simulink model "sptr"  (R2026a)
settings: Solver=daessc  StopTime=simlength  FixedStep=Ts  MaxStep=Ts  RelTol=Ts  AbsTol=Ts  EnableMultiTasking=on
values from neighbouring files (symbols this model uses):
  I_FS = Iout_dc_nom * margin_factor    (= 103.5)    [init_model.m]
  kgrid = 1    [init_model.m]
  LFu_dc = 1.2e-3    (= 0.0012)    [init_model.m]
  pll_i1 = 80    [init_model.m]
  pll_p = 1    [init_model.m]
  RLFu_dc = 2e-4    (= 0.0002)    [init_model.m]
  Rload = 1.2/4    (= 0.3)    [init_model.m]
  Tcontrol_rect = tPWM_RECT    (= 0.0002)    [init_model.m]
  Ts = Tc/1    (= 1e-05)    [init_model.m]
  V_FS = Vout_dc_nom * margin_factor    (= 391)    [init_model.m]
  Vnom_ac_adc = 400/sqrt(3)*sqrt(2)    [init_model.m]
  Vphase1 = Vline1/sqrt(3)    [init_model.m]
  w_grid = f_grid*2*pi    (= 314.159265359)    [init_model.m]
undefined symbols (not defined in the file or in its folder): magnitude
libraries: fl_lib x137, nesl_utility x33, ee_lib x15, first_harmonic_tracker x3
(part 1 of 3)
settings Model: SimulationMode=accelerator  Creator=LTNBDA  LastModifiedBy=dbagn
settings SolverCC: ZeroCrossControl=EnableAll  ZeroCrossAlgorithm=Adaptive  SolverResetMethod=Robust
settings DataIOCC: MaxDataPoints=1  SignalLoggingSaveFormat=ModelDataLogs
settings OptimizationCC: InitFltsAndDblsToZero=on  EfficientMapNaN2IntZero=off
settings DebuggingCC: SaveWithParameterizedLinksMsg=none  SignalResolutionControl=TryResolveAllWithWarning  MultiTaskDSMMsg=warning  MultiTaskCondExecSysMsg=none
settings HardwareCC: ProdBitPerLong=64.0  ProdHWDeviceType=Generic->64-bit Embedded Processor (LP64)  TargetBitPerPointer=64.0  TargetBitPerSizeT=64.0  TargetBitPerPtrDiffT=64.0  TargetLongLongMode=on  TargetIntDivRoundTo=Zero  TargetEndianess=LittleEndian  TargetWordSize=64.0  TargetHWDeviceType=MATLAB Host  ProdEqTarget=off
settings SFSimCC: SimCustomHeaderCode=|
  | #include "math_f.h"
  | #include "mavgflt.h"
  | #include "mavgflt_simulink.h"
  | #include "bemf_obsv.h"
  | #include "bemf_obsv_simulink.h"
  | #include "bemf_obsv_load_est.h"
  | #include "bemf_obsv_load_est_simulink.h"
  | #include "dqvector_pi.h"
  | #include "dqvector_pi_simulink.h"
  | #include "sv_pwm_simulink.h"
  | #include "sv_pwm.h"
  | #include "six_pulse_rect.h"
  | #include "twelve_pulse_rect.h"
  | #include "first_harmonic_tracker.h"
  | #include "first_harmonic_tracker_simulink.h"
  | #include "dqpll_thyr.h"
  | #include "dqpll_thyr_simulink.h"
  | #include "dqpll_grid.h"
  | #include "dqpll_grid_simulink.h"
settings SFSimCC: SimUserSources=|
  | "mavgflt_simulink.c"
  | "mavgflt.c"
  | "bemf_obsv_simulink.c"
  | "bemf_obsv.c"
  | "bemf_obsv_load_est_simulink.c"
  | "bemf_obsv_load_est.c"
  | "dqvector_pi.c"
  | "dqvector_pi_simulink.c"
  | "sv_pwm_simulink.c"
  | "sv_pwm.c"
  | "six_pulse_rect.c"
  | "twelve_pulse_rect.c"
  | "first_harmonic_tracker_simulink.c"
  | "first_harmonic_tracker.c"
  | "dqpll_thyr_simulink.c"
  | "dqpll_thyr.c"
  | "dqpll_grid_simulink.c"
  | "dqpll_grid.c"
settings SFSimCC: SimUserIncludeDirs=|
  | include
  | src
settings CodeAppCC: MaxIdLength=128.0
settings GRTTargetCC: CombineOutputUpdateFcns=off  GRTInterface=on
settings SimscapeCC: SimscapeNormalizeSystem=off  SimscapeNominalValues="[{\"value\":\"1\",\"unit\":\"A\"},{\"value\":\"1\",\"unit\":\"bar\"},{\"value\":\"1\",\"unit\":\"cm^2\"},{\"value\":\"1\",\"unit\":\"cm^3/s\"},{\"value\":\"1\",\"unit\":\"kJ/kg\"},{\"value\":\"1\",\"unit\":\"kW\"},{\"value\":\"1\",\"unit\":\"l\"},{\"value\":\"1\",\"unit\":\"N\"},{\"value\":\"1\",\"unit\":\"N*m\"},{\"value\":\"1\",\"unit\":\"V\"}]"  SimscapeLogType=none  SimscapeLogDataHistory=5000.0

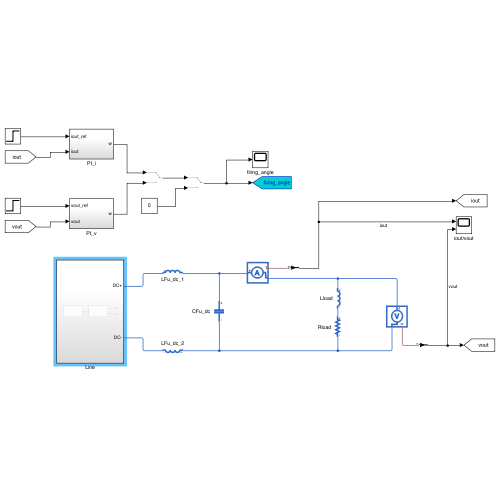
[thumbnail: Simulink's stored preview of the top-level diagram]
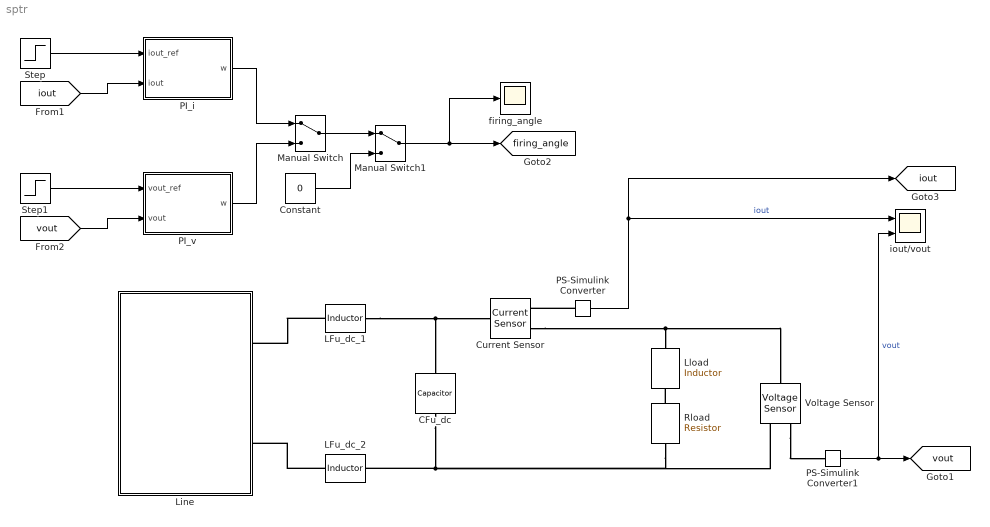
== system sptr ==
  CFu_dc : fl_lib/Electrical/Electrical Elements/Capacitor  c=CFu_dc F  r=RCFu_dc Ohm  g=0 1/Ohm  i_specify=off  i_priority=None  i=0 A  i_nominal_specify=off  i_nominal_value=1  i_nominal_unit=A  v_specify=off  v_priority=None  v=0 V  v_nominal_specify=off  v_nominal_value=1  v_nominal_unit=V  vc_specify=off  vc_priority=High  vc=0 V  vc_nominal_specify=off  vc_nominal_value=1  vc_nominal_unit=V
  Constant : Constant  Value=0
  Current Sensor : fl_lib/Electrical/Electrical Sensors/Current Sensor
  LFu_dc_1 : fl_lib/Electrical/Electrical Elements/Inductor  l=LFu_dc/2 H  r=RLFu_dc/2 Ohm  g=1e-9 1/Ohm  i_specify=off  i_priority=None  i=0 A  i_nominal_specify=off  i_nominal_value=1  i_nominal_unit=A  v_specify=off  v_priority=None  v=0 V  v_nominal_specify=off  v_nominal_value=1  v_nominal_unit=V  i_L_specify=off  i_L_priority=High  i_L=0 A  i_L_nominal_specify=off  i_L_nominal_value=1  i_L_nominal_unit=A
  LFu_dc_2 : fl_lib/Electrical/Electrical Elements/Inductor  l=LFu_dc/2 H  r=RLFu_dc/2 Ohm  g=1e-9 1/Ohm  i_specify=off  i_priority=None  i=0 A  i_nominal_specify=off  i_nominal_value=1  i_nominal_unit=A  v_specify=off  v_priority=None  v=0 V  v_nominal_specify=off  v_nominal_value=1  v_nominal_unit=V  i_L_specify=off  i_L_priority=High  i_L=0 A  i_L_nominal_specify=off  i_L_nominal_value=1  i_L_nominal_unit=A
  Line : Subsystem
  Lload : fl_lib/Electrical/Electrical Elements/Inductor  l=Lload H  r=0 Ohm  g=1e-9 1/Ohm  i_specify=off  i_priority=None  i=0 A  i_nominal_specify=off  i_nominal_value=1  i_nominal_unit=A  v_specify=off  v_priority=None  v=0 V  v_nominal_specify=off  v_nominal_value=1  v_nominal_unit=V  i_L_specify=off  i_L_priority=High  i_L=0 A  i_L_nominal_specify=off  i_L_nominal_value=1  i_L_nominal_unit=A
  Manual Switch : ManualSwitch
  Manual Switch1 : ManualSwitch
  PI_i : Subsystem
  PI_v : Subsystem
  PS-Simulink Converter : nesl_utility/PS-Simulink Converter  PhysicalDomain=network_engine_domain  SubClassName=ps_output  LeftPortType=input  RightPortType=output  PseudoPeriodic=off  Frequencies=[]  VectorFormat=1-D array  Unit=A  AffineConversion=off
  PS-Simulink Converter1 : nesl_utility/PS-Simulink Converter  PhysicalDomain=network_engine_domain  SubClassName=ps_output  LeftPortType=input  RightPortType=output  PseudoPeriodic=off  Frequencies=[]  VectorFormat=1-D array  Unit=V  AffineConversion=on
  Rload : fl_lib/Electrical/Electrical Elements/Resistor  R=Rload*2 Ohm  i_specify=off  i_priority=None  i=0 A  i_nominal_specify=off  i_nominal_value=1  i_nominal_unit=A  v_specify=off  v_priority=None  v=0 V  v_nominal_specify=off  v_nominal_value=1  v_nominal_unit=V
  Step : Step  Time=0.5  FinalValue=500/I_FS  SampleTime=0
  Step1 : Step  Time=0.5  FinalValue=200/V_FS  SampleTime=0
  Voltage Sensor : fl_lib/Electrical/Electrical Sensors/Voltage Sensor
  firing_angle : Scope
      settings: ActiveDisplayYMinimum=-0.39269908169872403  ActiveDisplayYMaximum=3.5342917352885173  DataLoggingVariableName=ScopeData5
  iout/vout : Scope  NumInputPorts=2
      settings: SampleTime=Tcontrol_rect  ActiveDisplayYMinimum=-109.3182  ActiveDisplayYMaximum=967.41622  DataLoggingVariableName=ScopeData10
  tag scope: firing_angle=global, iout=global, vout=global
  wires:
  PS-Simulink Converter/1 -> iout/vout/1, [iout]  "iout"
  Step/1 -> PI_i/1(iout_ref)
  PS-Simulink Converter1/1 -> iout/vout/2, [vout]  "vout"
  [iout] -> PI_i/2(iout)
  [vout] -> PI_v/2(vout)
  Step1/1 -> PI_v/1(vout_ref)
  PI_i/1(w) -> Manual Switch/1
  PI_v/1(w) -> Manual Switch/2
  Manual Switch/1 -> Manual Switch1/1
  Manual Switch1/1 -> firing_angle/1, [firing_angle]
  Constant/1 -> Manual Switch1/2
  connections:
  LFu_dc_1/RConn1 -- CFu_dc/LConn1 -- Current Sensor/LConn1
  CFu_dc/RConn1 -- Rload/RConn1 -- Voltage Sensor/RConn2 -- LFu_dc_2/LConn1
  LFu_dc_2/RConn1 -- Line/RConn2
  LFu_dc_1/LConn1 -- Line/RConn1
  Rload/LConn1 -- Lload/RConn1
  PS-Simulink Converter/LConn1 -- Current Sensor/RConn1
  Current Sensor/RConn2 -- Lload/LConn1 -- Voltage Sensor/LConn1
  Voltage Sensor/RConn1 -- PS-Simulink Converter1/LConn1

== system sptr/Line ==
  Grid : Subsystem
  six_pulse rectifier : Subsystem
  DC+ : PMIOPort  Side=Right
  DC- : PMIOPort  Port=2  Side=Right
  connections:
  six_pulse rectifier/RConn1 -- DC+/RConn1
  Grid/RConn1 -- six_pulse rectifier/LConn1
  six_pulse rectifier/RConn2 -- DC-/RConn1

== system sptr/PI_i ==
  iout_ref : Inport
  iout : Inport  Port=2
  1/Ti : Gain  Gain=0.15  SaturateOnIntegerOverflow=on  OutDataTypeStr=Inherit: Same as input  ParamDataTypeStr=Inherit: Same as input
  1/Ti2 : Gain  Gain=1/I_FS  SaturateOnIntegerOverflow=on  OutDataTypeStr=Inherit: Same as input  ParamDataTypeStr=Inherit: Same as input
  Saturation : Saturate  UpperLimit=pi  LowerLimit=0.1
  Saturation1 : Saturate  UpperLimit=1  LowerLimit=-1
  Sum1 : Sum  Inputs=+++  SaturateOnIntegerOverflow=on
  Sum2 : Sum  Inputs=+-  SaturateOnIntegerOverflow=on
  Sum3 : Sum  Inputs=-+  SaturateOnIntegerOverflow=on
  Trigonometric Function : Trigonometry  Operator=acos
  Unit Delay1 : UnitDelay  SampleTime=Tcontrol_rect
  Unit Delay4 : UnitDelay  SampleTime=Tcontrol_rect
  kp : Gain  Gain=8*Tcontrol_rect  SaturateOnIntegerOverflow=on  OutDataTypeStr=Inherit: Same as input  ParamDataTypeStr=Inherit: Same as input
  w : Outport  VectorParamsAs1DForOutWhenUnconnected=off
  wires:
  Sum2/1 -> 1/Ti/1, kp/1
  kp/1 -> Sum1/2
  1/Ti/1 -> Sum3/1, Sum1/1
  Unit Delay4/1 -> Sum1/3
  Sum3/1 -> Unit Delay4/1
  Sum1/1 -> Saturation1/1
  Saturation/1 -> Unit Delay1/1
  iout/1 -> 1/Ti2/1
  iout_ref/1 -> Sum2/1
  1/Ti2/1 -> Sum2/2
  Unit Delay1/1 -> w/1
  Saturation1/1 -> Sum3/2, Trigonometric Function/1
  Trigonometric Function/1 -> Saturation/1

== system sptr/PI_v ==
  vout_ref : Inport
  vout : Inport  Port=2
  1/Ti : Gain  Gain=0.5  SaturateOnIntegerOverflow=on  OutDataTypeStr=Inherit: Same as input  ParamDataTypeStr=Inherit: Same as input
  1/Ti2 : Gain  Gain=1/V_FS  SaturateOnIntegerOverflow=on  OutDataTypeStr=Inherit: Same as input  ParamDataTypeStr=Inherit: Same as input
  Saturation : Saturate  UpperLimit=pi  LowerLimit=0
  Saturation1 : Saturate  UpperLimit=1  LowerLimit=-1
  Sum1 : Sum  Inputs=+++  SaturateOnIntegerOverflow=on
  Sum2 : Sum  Inputs=+-  SaturateOnIntegerOverflow=on
  Sum3 : Sum  Inputs=-+  SaturateOnIntegerOverflow=on
  Trigonometric Function : Trigonometry  Operator=acos
  Unit Delay1 : UnitDelay  SampleTime=Tcontrol_rect
  Unit Delay4 : UnitDelay  SampleTime=Tcontrol_rect
  kp : Gain  Gain=18*Tcontrol_rect  SaturateOnIntegerOverflow=on  OutDataTypeStr=Inherit: Same as input  ParamDataTypeStr=Inherit: Same as input
  w : Outport  VectorParamsAs1DForOutWhenUnconnected=off
  wires:
  Trigonometric Function/1 -> Saturation/1
  Saturation1/1 -> Trigonometric Function/1, Sum3/2
  Unit Delay1/1 -> w/1
  1/Ti2/1 -> Sum2/2
  vout_ref/1 -> Sum2/1
  vout/1 -> 1/Ti2/1
  Saturation/1 -> Unit Delay1/1
  Sum1/1 -> Saturation1/1
  Sum3/1 -> Unit Delay4/1
  Unit Delay4/1 -> Sum1/3
  1/Ti/1 -> Sum1/1, Sum3/1
  kp/1 -> Sum1/2
  Sum2/1 -> kp/1, 1/Ti/1

== system sptr/Line/Grid ==
  Controlled Voltage Source : fl_lib/Electrical/Electrical Sources/Controlled Voltage Source
  Controlled Voltage Source1 : fl_lib/Electrical/Electrical Sources/Controlled Voltage Source
  Controlled Voltage Source2 : fl_lib/Electrical/Electrical Sources/Controlled Voltage Source
  Electrical Reference : fl_lib/Electrical/Electrical Elements/Electrical Reference
  LV mains : Subsystem
  Phase Splitter : ee_lib/Connectors & References/Phase Splitter
  Simulink-PS Converter : nesl_utility/Simulink-PS Converter  PhysicalDomain=network_engine_domain  SubClassName=ps_input  LeftPortType=input  RightPortType=output  PseudoPeriodic=off  Frequencies=[]  NoiseDistribution=none  NoiseParameters=[]  Unit=V  AffineConversion=on  FilteringAndDerivatives=provide  SimscapeFilterOrder=1  InputFilterTimeConstant=0.001  UdotUserProvided=0
  Simulink-PS Converter1 : nesl_utility/Simulink-PS Converter  PhysicalDomain=network_engine_domain  SubClassName=ps_input  LeftPortType=input  RightPortType=output  PseudoPeriodic=off  Frequencies=[]  NoiseDistribution=none  NoiseParameters=[]  Unit=V  AffineConversion=on  FilteringAndDerivatives=provide  SimscapeFilterOrder=1  InputFilterTimeConstant=0.001  UdotUserProvided=0
  Simulink-PS Converter2 : nesl_utility/Simulink-PS Converter  PhysicalDomain=network_engine_domain  SubClassName=ps_input  LeftPortType=input  RightPortType=output  PseudoPeriodic=off  Frequencies=[]  NoiseDistribution=none  NoiseParameters=[]  Unit=V  AffineConversion=on  FilteringAndDerivatives=provide  SimscapeFilterOrder=1  InputFilterTimeConstant=0.001  UdotUserProvided=0
  Solver Configuration : nesl_utility/Solver Configuration  PhysicalDomain=network_engine_domain  SubClassName=solver  LeftPortType=input  RightPortType=generic  Tones=[]  Harmonics=[]  SimulateNoise=off  Profile=off  UseLocalSampling=off  EnableSwitchedLinearOptims=on  FrequencyDomain=off  UseCCode=off  RelTol=0.001  AbsTol=1e-06  MinStep=1e-09  ToWorkspace=off  RevertToSquareIcSolve=off  NumHomotopyIterations=100  PhasorMode=off  PhasorModeNumHarmonics=1  ConsistencySolver=NEWTON_FTOL  CanonicalOrdering=UNORDERED  OptimizeIntermediates=UNOPTIMIZED  IndexReductionMethod=DerivativeReplacement  DoDC=off  ResidualTolerance=1e-09  ConsistencyTolSource=GLOBAL  ConsistencyAbsTol=0.001  ConsistencyRelTol=0.001  ConsistencyTolFactor=0.001  UseLocalSolver=on  LocalSolverChoice=NE_BACKWARD_EULER_ADVANCER  ResolveIndetEquations=on  FunctionEvalNumThread=1  LocalSolverSampleTime=Tcontrol_rect  DoFixedCost=on  MaxNonlinIter=3  MaxModeIter=2  ComputeImpulses=off  ImpulseIterations=2  LinearAlgebra=auto  LinearAlgebraNumThread=0  EquationFormulation=NE_TIME_EF  DelaysMemoryBudget=1024  AutomaticFiltering=on  FilteringTimeConstant=0.001  PartitionStorageMethod=AS_NEEDED  PartitionMemoryBudget=1024  PartitionMethod=ROBUST  MultibodyUseLocalSolver=off  MultibodyLocalSolverChoice=ODE1  MultibodyLocalSolverSampleTime=0.001
  Two-Winding Transformer (Three-Phase) : ee_lib/Passive/Transformers/Two-Winding Transformer (Three-Phase)  SRated=1500e3 A*V  FRated=50 Hz  Winding1Connection=ee.enum.windingconnection.delta1  VRated1=400 V  Winding2Connection=ee.enum.windingconnection.Y  VRated2=400 V  CoreType=ee.enum.coretype.threelimb  pu_Rw1=0.02  pu_Rw2=0.02  leakage_reactance_option=ee.enum.transformer_leakage.include  pu_Xl1=0.05  pu_Xl2=0.05  magnetizing_resistance_option=ee.enum.transformer_magnetizingResistance.exclude  pu_Rm=500  magnetizing_reactance_option=ee.enum.transformer_magnetizingReactance.exclude  saturation_option=ee.enum.transformer_saturation.exclude  pu_Xm=500  current_data=[0, .002, 1, 2]  magnetic_flux_data=[0, 1.2, 1.5, 1.51]  pu_X0=0.5  i1_specify=off  i1_priority=None  i1=[0, 0, 0] A  i1_nominal_specify=off  i1_nominal_value=1  i1_nominal_unit=A  i2_specify=off  i2_priority=None  i2=[0, 0, 0] A  i2_nominal_specify=off  i2_nominal_value=1  i2_nominal_unit=A  phi_specify=off  phi_priority=None  phi=[0, 0, 0]  phi_nominal_specify=off  phi_nominal_value=1  phi_nominal_unit=1
  ui/line : Scope  NumInputPorts=2
      settings: SampleTime=Tcontrol_rect  ActiveDisplayYMinimum=-1.25  ActiveDisplayYMaximum=1.25
  voltage_measure3 : Subsystem
  grid_line : PMIOPort  Side=Right
  wires:
  voltage_measure3/2(iabc_line) -> ui/line/2
  LV mains/1(Vma) -> Simulink-PS Converter/1
  LV mains/3(Vmc) -> Simulink-PS Converter2/1
  LV mains/2(Vmb) -> Simulink-PS Converter1/1
  voltage_measure3/1(grid_line) -> ui/line/1
  connections:
  Controlled Voltage Source1/LConn1 -- voltage_measure3/LConn2
  Phase Splitter/LConn1 -- Two-Winding Transformer (Three-Phase)/LConn1
  Controlled Voltage Source/RConn1 -- Simulink-PS Converter/RConn1
  Controlled Voltage Source2/RConn2 -- Controlled Voltage Source/RConn2 -- Controlled Voltage Source1/RConn2 -- Solver Configuration/RConn1 -- Electrical Reference/LConn1
  voltage_measure3/RConn2 -- Phase Splitter/RConn2
  Controlled Voltage Source2/LConn1 -- voltage_measure3/LConn3
  voltage_measure3/RConn3 -- Phase Splitter/RConn3
  Controlled Voltage Source1/RConn1 -- Simulink-PS Converter1/RConn1
  Controlled Voltage Source2/RConn1 -- Simulink-PS Converter2/RConn1
  Controlled Voltage Source/LConn1 -- voltage_measure3/LConn1
  voltage_measure3/RConn1 -- Phase Splitter/RConn1
  Two-Winding Transformer (Three-Phase)/RConn1 -- grid_line/RConn1

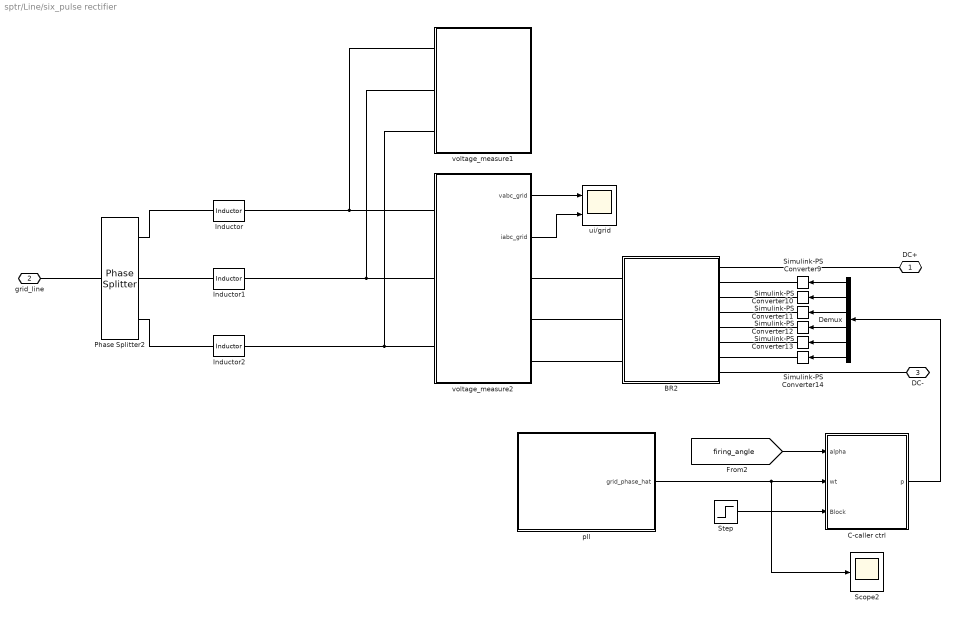
== system sptr/Line/six_pulse rectifier ==
  BR2 : Subsystem
  C-caller ctrl : Subsystem
  Demux : Demux  Outputs=6
  Inductor : fl_lib/Electrical/Electrical Elements/Inductor  l=65e-6 H  r=0 Ohm  g=1e-9 1/Ohm  i_specify=off  i_priority=None  i=0 A  i_nominal_specify=off  i_nominal_value=1  i_nominal_unit=A  v_specify=off  v_priority=None  v=0 V  v_nominal_specify=off  v_nominal_value=1  v_nominal_unit=V  i_L_specify=off  i_L_priority=High  i_L=0 A  i_L_nominal_specify=off  i_L_nominal_value=1  i_L_nominal_unit=A
  Inductor1 : fl_lib/Electrical/Electrical Elements/Inductor  l=65e-6 H  r=0 Ohm  g=1e-9 1/Ohm  i_specify=off  i_priority=None  i=0 A  i_nominal_specify=off  i_nominal_value=1  i_nominal_unit=A  v_specify=off  v_priority=None  v=0 V  v_nominal_specify=off  v_nominal_value=1  v_nominal_unit=V  i_L_specify=off  i_L_priority=High  i_L=0 A  i_L_nominal_specify=off  i_L_nominal_value=1  i_L_nominal_unit=A
  Inductor2 : fl_lib/Electrical/Electrical Elements/Inductor  l=65e-6 H  r=0 Ohm  g=1e-9 1/Ohm  i_specify=off  i_priority=None  i=0 A  i_nominal_specify=off  i_nominal_value=1  i_nominal_unit=A  v_specify=off  v_priority=None  v=0 V  v_nominal_specify=off  v_nominal_value=1  v_nominal_unit=V  i_L_specify=off  i_L_priority=High  i_L=0 A  i_L_nominal_specify=off  i_L_nominal_value=1  i_L_nominal_unit=A
  Phase Splitter2 : ee_lib/Connectors & References/Phase Splitter
  Scope2 : Scope
      settings: SampleTime=Tcontrol_rect  ActiveDisplayYMinimum=-0.78135  ActiveDisplayYMaximum=6.5313
  Simulink-PS Converter{9..10,12..14} (5 alike) : nesl_utility/Simulink-PS Converter  PhysicalDomain=network_engine_domain  SubClassName=ps_input  LeftPortType=input  RightPortType=output  PseudoPeriodic=off  Frequencies=[]  NoiseDistribution=none  NoiseParameters=[]  Unit=V  AffineConversion=on  FilteringAndDerivatives=provide  SimscapeFilterOrder=1  InputFilterTimeConstant=0.001  UdotUserProvided=0
  Simulink-PS Converter11 : nesl_utility/Simulink-PS Converter  PhysicalDomain=network_engine_domain  SubClassName=ps_input  LeftPortType=input  RightPortType=output  PseudoPeriodic=off  Frequencies=[]  NoiseDistribution=none  NoiseParameters=[]  Unit=V  AffineConversion=off  FilteringAndDerivatives=provide  SimscapeFilterOrder=1  InputFilterTimeConstant=0.001  UdotUserProvided=0
  Step : Step  Time=0.25  InitialValue=1  FinalValue=0  SampleTime=Tcontrol_rect
  pll : Subsystem
  ui/grid : Scope  NumInputPorts=2
      settings: SampleTime=Tcontrol_rect  ActiveDisplayYMinimum=-1.2499998689252119  ActiveDisplayYMaximum=1.2499998689252119
  voltage_measure1 : Subsystem
  voltage_measure2 : Subsystem
  DC+ : PMIOPort  Side=Right
  grid_line : PMIOPort  Port=2  Side=Left
  DC- : PMIOPort  Port=3  Side=Right
  wires:
  C-caller ctrl/1(p) -> Demux/1
  voltage_measure2/1(vabc_grid) -> ui/grid/1
  Demux/2 -> Simulink-PS Converter10/1
  Step/1 -> C-caller ctrl/3(Block)
  Demux/4 -> Simulink-PS Converter12/1
  pll/1(grid_phase_hat) -> Scope2/1, C-caller ctrl/2(wt)
  Demux/1 -> Simulink-PS Converter9/1
  [firing_angle] -> C-caller ctrl/1(alpha)
  Demux/5 -> Simulink-PS Converter13/1
  Demux/6 -> Simulink-PS Converter14/1
  Demux/3 -> Simulink-PS Converter11/1
  voltage_measure2/2(iabc_grid) -> ui/grid/2
  connections:
  voltage_measure2/RConn1 -- BR2/RConn1
  BR2/LConn3 -- Simulink-PS Converter10/RConn1
  BR2/LConn7 -- Simulink-PS Converter14/RConn1
  grid_line/RConn1 -- Phase Splitter2/LConn1
  BR2/LConn6 -- Simulink-PS Converter13/RConn1
  voltage_measure1/LConn2 -- Inductor1/RConn1 -- voltage_measure2/LConn2
  BR2/LConn2 -- Simulink-PS Converter9/RConn1
  BR2/LConn5 -- Simulink-PS Converter12/RConn1
  voltage_measure1/LConn3 -- Inductor2/RConn1 -- voltage_measure2/LConn3
  BR2/LConn8 -- DC-/RConn1
  voltage_measure2/RConn3 -- BR2/RConn3
  BR2/LConn4 -- Simulink-PS Converter11/RConn1
  voltage_measure1/LConn1 -- Inductor/RConn1 -- voltage_measure2/LConn1
  voltage_measure2/RConn2 -- BR2/RConn2
  BR2/LConn1 -- DC+/RConn1
  Phase Splitter2/RConn1 -- Inductor/LConn1
  Phase Splitter2/RConn2 -- Inductor1/LConn1
  Phase Splitter2/RConn3 -- Inductor2/LConn1

== system sptr/Line/Grid/LV mains ==
  Clock : Clock
  Constant2 : Constant  Value=2*pi/3
  Constant3 : Constant  Value=4*pi/3
  Gain : Gain  Gain=w_grid
  Gain1 : Gain  Gain=Vphase1*sqrt(2)
  Gain2 : Gain  Gain=Vphase1*sqrt(2)
  Gain3 : Gain  Gain=Vphase1*sqrt(2)
  Gain4 : Gain  Gain=kgrid
  Gain5 : Gain  Gain=kgrid
  Gain6 : Gain  Gain=kgrid
  Sum2 : Sum  Inputs=+-|
  Sum3 : Sum  Inputs=+-|
  Trigonometric Function : Trigonometry  Operator=cos
  Trigonometric Function1 : Trigonometry  Operator=cos
  Trigonometric Function2 : Trigonometry  Operator=cos
  Vma : Outport
  Vmb : Outport  Port=2
  Vmc : Outport  Port=3
  wires:
  Trigonometric Function/1 -> Gain1/1
  Constant2/1 -> Sum2/2
  Sum2/1 -> Trigonometric Function1/1
  Constant3/1 -> Sum3/2
  Sum3/1 -> Trigonometric Function2/1
  Clock/1 -> Gain/1
  Gain/1 -> Sum3/1, Trigonometric Function/1, Sum2/1  "wt"
  Trigonometric Function1/1 -> Gain2/1
  Trigonometric Function2/1 -> Gain3/1
  Gain1/1 -> Gain4/1
  Gain2/1 -> Gain5/1
  Gain3/1 -> Gain6/1
  Gain4/1 -> Vma/1
  Gain5/1 -> Vmb/1
  Gain6/1 -> Vmc/1

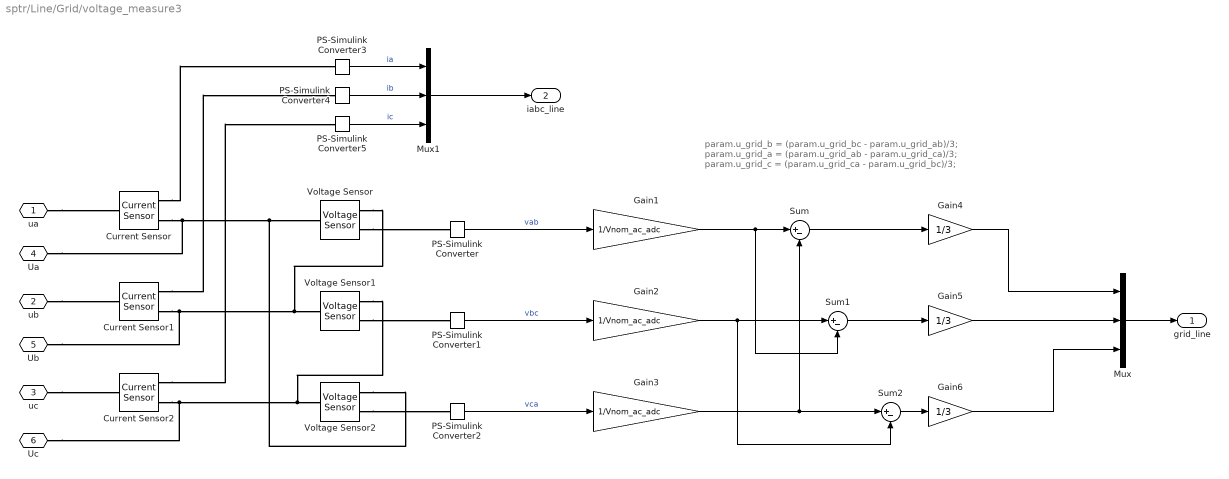
== system sptr/Line/Grid/voltage_measure3 ==
  note: param.u_grid_b = (param.u_grid_bc - param.u_grid_ab)/3;
      | 	param.u_grid_a = (param.u_grid_ab - param.u_grid_ca)/3;
      | 	param.u_grid_c = (param.u_grid_ca - param.u_grid_bc)/3;
  Current Sensor : fl_lib/Electrical/Electrical Sensors/Current Sensor
  Current Sensor1 : fl_lib/Electrical/Electrical Sensors/Current Sensor
  Current Sensor2 : fl_lib/Electrical/Electrical Sensors/Current Sensor
  Gain1 : Gain  Gain=1/Vnom_ac_adc
  Gain2 : Gain  Gain=1/Vnom_ac_adc
  Gain3 : Gain  Gain=1/Vnom_ac_adc
  Gain4 : Gain  Gain=1/3
  Gain5 : Gain  Gain=1/3
  Gain6 : Gain  Gain=1/3
  Mux : Mux  Inputs=3
  Mux1 : Mux  Inputs=3
  PS-Simulink Converter : nesl_utility/PS-Simulink Converter  PhysicalDomain=network_engine_domain  SubClassName=ps_output  LeftPortType=input  RightPortType=output  PseudoPeriodic=off  Frequencies=[]  VectorFormat=1-D array  Unit=inherit  AffineConversion=off
  PS-Simulink Converter1 : nesl_utility/PS-Simulink Converter  PhysicalDomain=network_engine_domain  SubClassName=ps_output  LeftPortType=input  RightPortType=output  PseudoPeriodic=off  Frequencies=[]  VectorFormat=1-D array  Unit=inherit  AffineConversion=off
  PS-Simulink Converter2 : nesl_utility/PS-Simulink Converter  PhysicalDomain=network_engine_domain  SubClassName=ps_output  LeftPortType=input  RightPortType=output  PseudoPeriodic=off  Frequencies=[]  VectorFormat=1-D array  Unit=inherit  AffineConversion=off
  PS-Simulink Converter3 : nesl_utility/PS-Simulink Converter  PhysicalDomain=network_engine_domain  SubClassName=ps_output  LeftPortType=input  RightPortType=output  PseudoPeriodic=off  Frequencies=[]  VectorFormat=1-D array  Unit=A  AffineConversion=off
  PS-Simulink Converter4 : nesl_utility/PS-Simulink Converter  PhysicalDomain=network_engine_domain  SubClassName=ps_output  LeftPortType=input  RightPortType=output  PseudoPeriodic=off  Frequencies=[]  VectorFormat=1-D array  Unit=A  AffineConversion=off
  PS-Simulink Converter5 : nesl_utility/PS-Simulink Converter  PhysicalDomain=network_engine_domain  SubClassName=ps_output  LeftPortType=input  RightPortType=output  PseudoPeriodic=off  Frequencies=[]  VectorFormat=1-D array  Unit=A  AffineConversion=off
  Sum : Sum  Inputs=|+-
  Sum1 : Sum  Inputs=|+-
  Sum2 : Sum  Inputs=|+-
  Voltage Sensor : fl_lib/Electrical/Electrical Sensors/Voltage Sensor
  Voltage Sensor1 : fl_lib/Electrical/Electrical Sensors/Voltage Sensor
  Voltage Sensor2 : fl_lib/Electrical/Electrical Sensors/Voltage Sensor
  ua : PMIOPort  Side=Left
  ub : PMIOPort  Port=2  Side=Left
  uc : PMIOPort  Port=3  Side=Left
  Ua : PMIOPort  Port=4  Side=Right
  Ub : PMIOPort  Port=5  Side=Right
  Uc : PMIOPort  Port=6  Side=Right
  grid_line : Outport
  iabc_line : Outport  Port=2
  wires:
  PS-Simulink Converter5/1 -> Mux1/3  "ic"
  PS-Simulink Converter3/1 -> Mux1/1  "ia"
  PS-Simulink Converter4/1 -> Mux1/2  "ib"
  Mux1/1 -> iabc_line/1
  Gain6/1 -> Mux/3
  Gain5/1 -> Mux/2
  Gain4/1 -> Mux/1
  Gain2/1 -> Sum1/1, Sum2/2
  Sum2/1 -> Gain6/1
  Sum1/1 -> Gain5/1
  Sum/1 -> Gain4/1
  Gain3/1 -> Sum/2, Sum2/1
  Gain1/1 -> Sum/1, Sum1/2
  Mux/1 -> grid_line/1
  PS-Simulink Converter/1 -> Gain1/1  "vab"
  PS-Simulink Converter2/1 -> Gain3/1  "vca"
  PS-Simulink Converter1/1 -> Gain2/1  "vbc"
  connections:
  Current Sensor2/RConn1 -- PS-Simulink Converter5/LConn1
  Current Sensor1/RConn1 -- PS-Simulink Converter4/LConn1
  Current Sensor/RConn1 -- PS-Simulink Converter3/LConn1
  uc/RConn1 -- Current Sensor2/LConn1
  ub/RConn1 -- Current Sensor1/LConn1
  ua/RConn1 -- Current Sensor/LConn1
  Voltage Sensor1/RConn1 -- PS-Simulink Converter1/LConn1
  Uc/RConn1 -- Current Sensor2/RConn2 -- Voltage Sensor1/RConn2 -- Voltage Sensor2/LConn1
  Voltage Sensor2/RConn1 -- PS-Simulink Converter2/LConn1
  Voltage Sensor/RConn1 -- PS-Simulink Converter/LConn1
  Ua/RConn1 -- Current Sensor/RConn2 -- Voltage Sensor2/RConn2 -- Voltage Sensor/LConn1
  Ub/RConn1 -- Current Sensor1/RConn2 -- Voltage Sensor/RConn2 -- Voltage Sensor1/LConn1

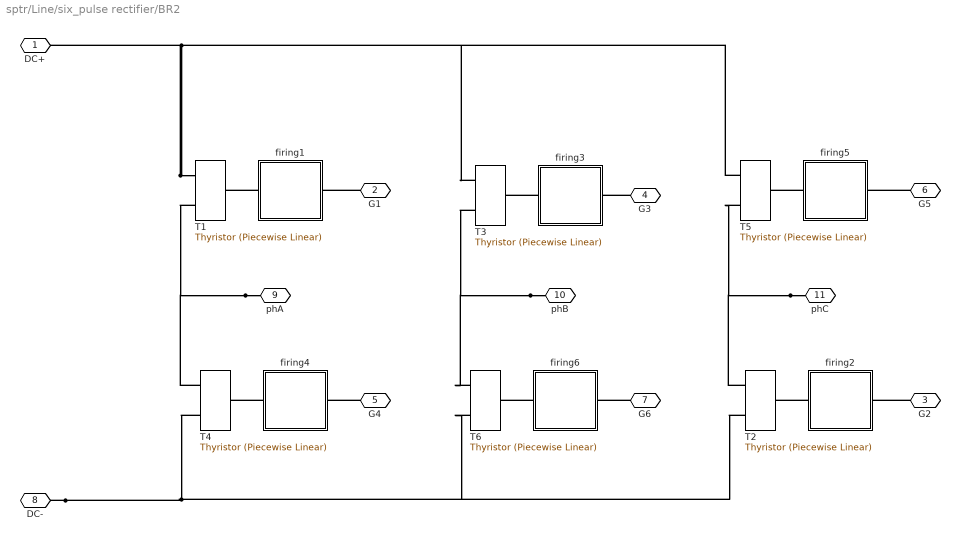
== system sptr/Line/six_pulse rectifier/BR2 ==
  T{1..6} (6 alike) : ee_lib/Semiconductors & Converters/Thyristor (Piecewise Linear)  port_option=ee.enum.controlport.ps  Vf=0.8 V  Ron=0.001 Ohm  Goff=1e-5 1/Ohm  Vgt=6 V  Ih=1 A  diode_param=1  diode_Vf=0.8 V  diode_Ron=0.001 Ohm  diode_Goff=1e-5 1/Ohm  diode_C=50e-9 F  diode_iRM=-235 A  diode_iF=300 A  diode_idot=-50 A/us  diode_trr_param=1  diode_trr_factor=3  diode_trr=15 us  diode_Qrr=1500 s*uA  iak_specify=off  iak_priority=None  iak=0 A  iak_nominal_specify=off  iak_nominal_value=1  iak_nominal_unit=A  vak_specify=off  vak_priority=None  vak=0 V  vak_nominal_specify=off  vak_nominal_value=1  vak_nominal_unit=V  vgk_specify=off  vgk_priority=None  vgk=0 V  vgk_nominal_specify=off  vgk_nominal_value=1  vgk_nominal_unit=V  thermal_loss_option=2  Von_data=[0, 1.1, 1.3, 1.45, 1.75, 2.25, 2.7; 0, 1, 1.15, 1.35, 1.7, 2.35, 3] V  Tj=[298.15, 398.15] K  Iout_data=[0, 10, 50, 100, 200, 400, 600] A  Eon_data=[0, .29, 1.43, 2.86, 5.71, 13.14, 22.86; 0, .57, 2.63, 5.14, 10.29, 20.57, 30.29] * 1e-3 J  Tj_loss=[298.15, 398.15] K  Iout_data_loss=[0, .1, 1, 5, 10, 20, 40, 70, 100] A  Eon_scalar=22.86e-3 J  Eoff_natural_commutation=10e-3 J  Voff=300 V  Iout_scalar=600 A  onCurrentMeasDelay=1e-4 s  diodeModelType=ee.enum.converters.diodeModelType.pwl  diodeTableType=ee.enum.diode.tableType.IfMat  diode_IfMat=[.07, .12, .19, 1.75, 4.24, 7.32, 11.2; .16, .3, .72, 2.14, 4.02, 6.35, 9.12] A  diode_VfMat=[.9, 1.15, 1.25, 1.5, 1.75, 2.17, 2.6, 2.85; .58, .68, .75, 1.1, 1.38, 1.77, 2.27, 2.7] V  diode_TjVec=[25, 125] degC  diode_VfVec=[.5, .7, .9, 1.3, 1.7, 2.1, 2.5] V  diode_IfVec=[.1, .2, .5, 1, 2, 4, 7, 10] A  diode_rec_loss_model=ee.enum.diode.reverseRecoveryModel.fixed  diode_ErecVal=0 J  diode_scaleWithIandV=true  diode_ErecMat=zeros(2, 3) J  diode_TjrecVec=[298.15, 398.15] K  diode_IfrecVec=[.1, 1, 10] A  diode_IrecVal=10 A  diode_VrecVal=10 V  diode_tFilter=1 / 1000 / 100 s  thermal_network_parameterization=ee.enum.thermalNetworkTopology.external  Rth=[.08, .5] K/W  Rth_Cauer=[.08, .1, .5] K/W  Rth_Foster=[.08, .14, .22, .16] K/W  thermal_mass_parameterization=ee.enum.thermalNetwork.timeconstant  thermal_mass=[.01, .5] J/K  thermal_mass_Cauer=[.01, .1, .5] J/K  thermal_mass_Foster=[.001, .005, .05, .5] J/K  thermal_time_constant=[.001, .2] s  thermal_time_constant_Cauer=[.001, .1, .2] s  thermal_time_constant_Foster=[7e-05, .0007, .01, .08] s  thermal_mass_initial_temperatures=[25, 25] degC  thermal_mass_initial_temperatures_Cauer=[25, 25, 25] degC  junction_thermal_mass=0.01 J/K  Tvec_initial_Foster=[25, 25, 25, 25] degC  junction_temperature_specify=off  junction_temperature_priority=None  junction_temperature=25 degC  junction_temperature_nominal_specify=off  junction_temperature_nominal_value=1  junction_temperature_nominal_unit=degC  Qj_specify=off  Qj_priority=None  Qj=0 W  Qj_nominal_specify=off  Qj_nominal_value=1  Qj_nominal_unit=W  accumulatedSwitchingLosses_specify=off  accumulatedSwitchingLosses_priority=None  accumulatedSwitchingLosses=0 J
  firing1 : Subsystem
  firing2 : Subsystem
  firing3 : Subsystem
  firing4 : Subsystem
  firing5 : Subsystem
  firing6 : Subsystem
  DC+ : PMIOPort  Side=Left
  G1 : PMIOPort  Port=2  Side=Left
  G2 : PMIOPort  Port=3  Side=Left
  G3 : PMIOPort  Port=4  Side=Left
  G4 : PMIOPort  Port=5  Side=Left
  G5 : PMIOPort  Port=6  Side=Left
  G6 : PMIOPort  Port=7  Side=Left
  DC- : PMIOPort  Port=8  Side=Left
  phA : PMIOPort  Port=9  Side=Right
  phB : PMIOPort  Port=10  Side=Right
  phC : PMIOPort  Port=11  Side=Right
  connections:
  firing6/RConn1 -- T6/LConn1
  firing5/RConn1 -- T5/LConn1
  firing4/RConn1 -- T4/LConn1
  firing3/RConn1 -- T3/LConn1
  firing2/RConn1 -- T2/LConn1
  firing1/RConn1 -- T1/LConn1
  G6/RConn1 -- firing6/LConn1
  G5/RConn1 -- firing5/LConn1
  G4/RConn1 -- firing4/LConn1
  G3/RConn1 -- firing3/LConn1
  G2/RConn1 -- firing2/LConn1
  G1/RConn1 -- firing1/LConn1
  DC-/RConn1 -- T4/RConn1 -- T6/RConn1 -- T2/RConn1
  phB/RConn1 -- T6/RConn2 -- T3/RConn1
  phC/RConn1 -- T5/RConn1 -- T2/RConn2
  phA/RConn1 -- T4/RConn2 -- T1/RConn1
  T1/RConn2 -- T3/RConn2 -- T5/RConn2 -- DC+/RConn1

== system sptr/Line/six_pulse rectifier/C-caller ctrl ==
  alpha : Inport  SampleTime=Ts
  wt : Inport  Port=2  SampleTime=Ts
  Block : Inport  Port=3  SampleTime=Ts
  Data Type Conversion1 : DataTypeConversion  OutDataTypeStr=single  SaturateOnIntegerOverflow=off  RndMeth=Floor
  Data Type Conversion2 : DataTypeConversion  OutDataTypeStr=single  SaturateOnIntegerOverflow=off  RndMeth=Floor
  Data Type Conversion4 : DataTypeConversion  OutDataTypeStr=int32  SaturateOnIntegerOverflow=off  RndMeth=Floor
  Zero-Order Hold1 : ZeroOrderHold  SampleTime=Tcontrol_rect
  Zero-Order Hold2 : ZeroOrderHold  SampleTime=Tcontrol_rect
  Zero-Order Hold3 : ZeroOrderHold  SampleTime=Tcontrol_rect
  ccaller : CCaller  FunctionName=sprcProcessSimulink  PortSpecificationStruct="%)30     .    ( <   8    (     @         %    \"     0    !     0         %  0 \"0    $    _    07)G3F%M90  4&]R=$YA;64 4V-O<&4     26YD97@     5'EP90      4VEZ90      27-';&]B86P   X    P    !@    @    $          4    (     0    (    !         !   @!W=   #@   #     &    \"     0         !0    @    !     @    $         $  \" '=T   .    .     8    (    !          %    \"     $    %     0         0  ...(+2073 chars)"  SampleTime=Tcontrol_rect
  pulses : Scope  NumInputPorts=4
      settings: SampleTime=Tc  ActiveDisplayYMinimum=-1.4999999999999996  ActiveDisplayYMaximum=13.5  DataLoggingVariableName=ScopeData2
  shift_level : Subsystem
  p : Outport  SampleTime=Ts  InitialOutput=0  VectorParamsAs1DForOutWhenUnconnected=off
  wires:
  alpha/1 -> Data Type Conversion2/1
  wt/1 -> Data Type Conversion1/1
  Data Type Conversion2/1 -> Zero-Order Hold2/1
  Data Type Conversion1/1 -> Zero-Order Hold3/1
  Data Type Conversion4/1 -> Zero-Order Hold1/1
  Zero-Order Hold3/1 -> pulses/2, ccaller/1  "phase"
  Zero-Order Hold2/1 -> pulses/3, ccaller/2  "firing_angle"
  Zero-Order Hold1/1 -> ccaller/3
  Block/1 -> Data Type Conversion4/1
  shift_level/1(PY) -> p/1, pulses/1  "p"
  ccaller/1 -> shift_level/1("PY ")
  [grid_voltage_filtered] -> pulses/4

== system sptr/Line/six_pulse rectifier/pll ==
  Bus Creator : BusCreator  Inputs=2
  Bus Selector : BusSelector  OutputSignals=phase_hat
  dqpll_thyr_ccaller : Subsystem
  dqpll_thyr_ccaller_s : Scope
      settings: ActiveDisplayYMinimum=-1.910201348364353  ActiveDisplayYMaximum=7.1920475736260414
  grid_phase_hats : Scope
      settings: ActiveDisplayYMinimum=-0.78537  ActiveDisplayYMaximum=7.06836  DataLoggingVariableName=ScopeData2
  pll_stageA : Subsystem
  pll_stageB : Subsystem
  grid_phase_hat : Outport
  wires:
  pll_stageA/1(Vgrid_a) -> pll_stageB/1(Vgrid_a)
  pll_stageA/2(Vgrid_b) -> pll_stageB/2(Vgrid_b)
  [vabc_grid_A] -> pll_stageA/1(ug)
  pll_stageB/1(wt_grid) -> Bus Creator/2  "grid_phase_hat_simulink"
  Bus Creator/1 -> grid_phase_hats/1
  dqpll_thyr_ccaller/1(m) -> dqpll_thyr_ccaller_s/1, Bus Selector/1
  Bus Selector/1 -> Bus Creator/1, grid_phase_hat/1  "<phase_hat>"

== system sptr/Line/six_pulse rectifier/voltage_measure1 ==
  Gain4 : Gain  Gain=1/3
  Gain5 : Gain  Gain=1/3
  Gain6 : Gain  Gain=1/3
  Mux : Mux  Inputs=3
  PS-Simulink Converter : nesl_utility/PS-Simulink Converter  PhysicalDomain=network_engine_domain  SubClassName=ps_output  LeftPortType=input  RightPortType=output  PseudoPeriodic=off  Frequencies=[]  VectorFormat=1-D array  Unit=inherit  AffineConversion=off
  PS-Simulink Converter1 : nesl_utility/PS-Simulink Converter  PhysicalDomain=network_engine_domain  SubClassName=ps_output  LeftPortType=input  RightPortType=output  PseudoPeriodic=off  Frequencies=[]  VectorFormat=1-D array  Unit=inherit  AffineConversion=off
  PS-Simulink Converter2 : nesl_utility/PS-Simulink Converter  PhysicalDomain=network_engine_domain  SubClassName=ps_output  LeftPortType=input  RightPortType=output  PseudoPeriodic=off  Frequencies=[]  VectorFormat=1-D array  Unit=inherit  AffineConversion=off
  Sum : Sum  Inputs=|+-
  Sum1 : Sum  Inputs=|+-
  Sum2 : Sum  Inputs=|+-
  Voltage Sensor : fl_lib/Electrical/Electrical Sensors/Voltage Sensor
  Voltage Sensor1 : fl_lib/Electrical/Electrical Sensors/Voltage Sensor
  Voltage Sensor2 : fl_lib/Electrical/Electrical Sensors/Voltage Sensor
  va : PMIOPort  Side=Left
  vb : PMIOPort  Port=2  Side=Left
  vc : PMIOPort  Port=3  Side=Left
  tag scope: vabc_grid_A=global
  wires:
  Mux/1 -> [vabc_grid_A]
  Gain6/1 -> Mux/3
  Gain4/1 -> Mux/1
  Gain5/1 -> Mux/2
  PS-Simulink Converter/1 -> Sum/1, Sum1/2
  Sum/1 -> Gain4/1
  PS-Simulink Converter2/1 -> Sum2/1, Sum/2
  Sum1/1 -> Gain5/1
  PS-Simulink Converter1/1 -> Sum2/2, Sum1/1
  Sum2/1 -> Gain6/1
  connections:
  Voltage Sensor/LConn1 -- Voltage Sensor2/RConn2 -- va/RConn1
  vb/RConn1 -- Voltage Sensor1/LConn1 -- Voltage Sensor/RConn2
  Voltage Sensor/RConn1 -- PS-Simulink Converter/LConn1
  Voltage Sensor1/RConn1 -- PS-Simulink Converter1/LConn1
  Voltage Sensor1/RConn2 -- Voltage Sensor2/LConn1 -- vc/RConn1
  Voltage Sensor2/RConn1 -- PS-Simulink Converter2/LConn1

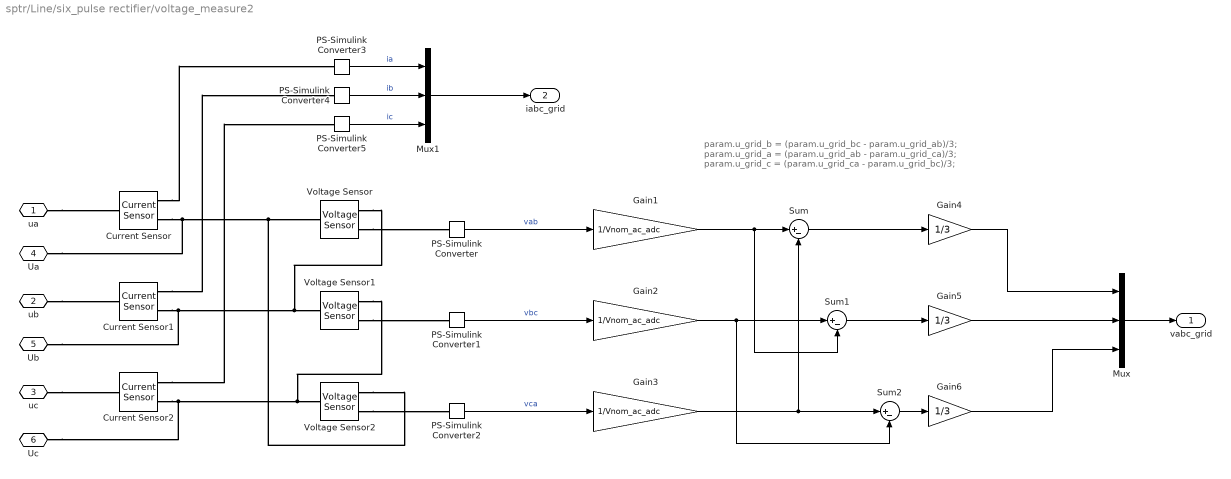
== system sptr/Line/six_pulse rectifier/voltage_measure2 ==
  note: param.u_grid_b = (param.u_grid_bc - param.u_grid_ab)/3;
      | 	param.u_grid_a = (param.u_grid_ab - param.u_grid_ca)/3;
      | 	param.u_grid_c = (param.u_grid_ca - param.u_grid_bc)/3;
  Current Sensor : fl_lib/Electrical/Electrical Sensors/Current Sensor
  Current Sensor1 : fl_lib/Electrical/Electrical Sensors/Current Sensor
  Current Sensor2 : fl_lib/Electrical/Electrical Sensors/Current Sensor
  Gain1 : Gain  Gain=1/Vnom_ac_adc
  Gain2 : Gain  Gain=1/Vnom_ac_adc
  Gain3 : Gain  Gain=1/Vnom_ac_adc
  Gain4 : Gain  Gain=1/3
  Gain5 : Gain  Gain=1/3
  Gain6 : Gain  Gain=1/3
  Mux : Mux  Inputs=3
  Mux1 : Mux  Inputs=3
  PS-Simulink Converter : nesl_utility/PS-Simulink Converter  PhysicalDomain=network_engine_domain  SubClassName=ps_output  LeftPortType=input  RightPortType=output  PseudoPeriodic=off  Frequencies=[]  VectorFormat=1-D array  Unit=inherit  AffineConversion=off
  PS-Simulink Converter1 : nesl_utility/PS-Simulink Converter  PhysicalDomain=network_engine_domain  SubClassName=ps_output  LeftPortType=input  RightPortType=output  PseudoPeriodic=off  Frequencies=[]  VectorFormat=1-D array  Unit=inherit  AffineConversion=off
  PS-Simulink Converter2 : nesl_utility/PS-Simulink Converter  PhysicalDomain=network_engine_domain  SubClassName=ps_output  LeftPortType=input  RightPortType=output  PseudoPeriodic=off  Frequencies=[]  VectorFormat=1-D array  Unit=inherit  AffineConversion=off
  PS-Simulink Converter3 : nesl_utility/PS-Simulink Converter  PhysicalDomain=network_engine_domain  SubClassName=ps_output  LeftPortType=input  RightPortType=output  PseudoPeriodic=off  Frequencies=[]  VectorFormat=1-D array  Unit=A  AffineConversion=off
  PS-Simulink Converter4 : nesl_utility/PS-Simulink Converter  PhysicalDomain=network_engine_domain  SubClassName=ps_output  LeftPortType=input  RightPortType=output  PseudoPeriodic=off  Frequencies=[]  VectorFormat=1-D array  Unit=A  AffineConversion=off
  PS-Simulink Converter5 : nesl_utility/PS-Simulink Converter  PhysicalDomain=network_engine_domain  SubClassName=ps_output  LeftPortType=input  RightPortType=output  PseudoPeriodic=off  Frequencies=[]  VectorFormat=1-D array  Unit=A  AffineConversion=off
  Sum : Sum  Inputs=|+-
  Sum1 : Sum  Inputs=|+-
  Sum2 : Sum  Inputs=|+-
  Voltage Sensor : fl_lib/Electrical/Electrical Sensors/Voltage Sensor
  Voltage Sensor1 : fl_lib/Electrical/Electrical Sensors/Voltage Sensor
  Voltage Sensor2 : fl_lib/Electrical/Electrical Sensors/Voltage Sensor
  ua : PMIOPort  Side=Left
  ub : PMIOPort  Port=2  Side=Left
  uc : PMIOPort  Port=3  Side=Left
  Ua : PMIOPort  Port=4  Side=Right
  Ub : PMIOPort  Port=5  Side=Right
  Uc : PMIOPort  Port=6  Side=Right
  vabc_grid : Outport
  iabc_grid : Outport  Port=2
  wires:
  PS-Simulink Converter1/1 -> Gain2/1  "vbc"
  PS-Simulink Converter2/1 -> Gain3/1  "vca"
  PS-Simulink Converter/1 -> Gain1/1  "vab"
  Mux/1 -> vabc_grid/1
  Gain1/1 -> Sum1/2, Sum/1
  Gain3/1 -> Sum2/1, Sum/2
  Sum/1 -> Gain4/1
  Sum1/1 -> Gain5/1
  Sum2/1 -> Gain6/1
  Gain2/1 -> Sum2/2, Sum1/1
  Gain4/1 -> Mux/1
  Gain5/1 -> Mux/2
  Gain6/1 -> Mux/3
  Mux1/1 -> iabc_grid/1
  PS-Simulink Converter4/1 -> Mux1/2  "ib"
  PS-Simulink Converter3/1 -> Mux1/1  "ia"
  PS-Simulink Converter5/1 -> Mux1/3  "ic"
  connections:
  Voltage Sensor/RConn2 -- Ub/RConn1 -- Current Sensor1/RConn2 -- Voltage Sensor1/LConn1
  Voltage Sensor2/RConn2 -- Ua/RConn1 -- Current Sensor/RConn2 -- Voltage Sensor/LConn1
  Voltage Sensor/RConn1 -- PS-Simulink Converter/LConn1
  Voltage Sensor2/RConn1 -- PS-Simulink Converter2/LConn1
  Voltage Sensor1/RConn2 -- Uc/RConn1 -- Current Sensor2/RConn2 -- Voltage Sensor2/LConn1
  Voltage Sensor1/RConn1 -- PS-Simulink Converter1/LConn1
  ua/RConn1 -- Current Sensor/LConn1
  ub/RConn1 -- Current Sensor1/LConn1
  uc/RConn1 -- Current Sensor2/LConn1
  Current Sensor/RConn1 -- PS-Simulink Converter3/LConn1
  Current Sensor1/RConn1 -- PS-Simulink Converter4/LConn1
  Current Sensor2/RConn1 -- PS-Simulink Converter5/LConn1
